simulink model "BIG_MUFF_PI_inputStage_ssc"  (R2025b)
settings: Solver=VariableStepAuto  StartTime=0  StopTime=5.1  FixedStep=1/96e3  RelTol=1e-3
libraries: fl_lib x17, ee_lib x11, nesl_utility x3
(part 2 of 2)

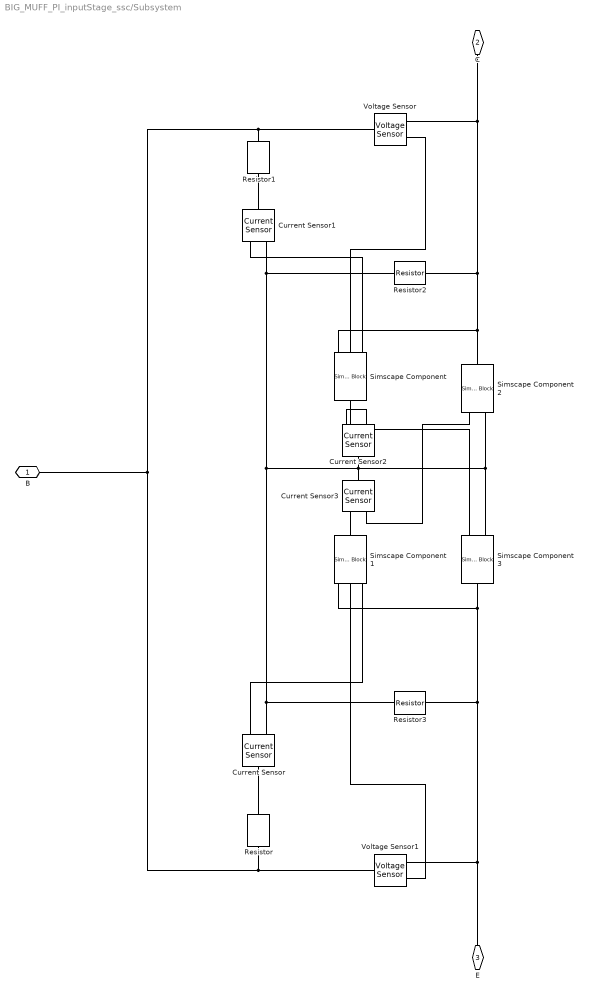
== system BIG_MUFF_PI_inputStage_ssc/Subsystem ==
  Current Sensor{,1..3} (4 alike) : fl_lib/Electrical/Electrical Sensors/Current Sensor
  Resistor : ee_lib/Passive/Resistor  R=1e-5 Ohm  enable_R_tol=0  R_tol=5  tol_distribution=1  nSigma=4  enable_operating_limits=0  operating_limit_action=2  power_rating=1 W  max_working_voltage=100 V  noise_mode=0  Tdevice=25 degC  sample_time=1e-3 s  repeatability=1  user_seed=0  auto_seed=418932850  power_derating_T1=70 degC  power_derating_T2=155 degC  operating_temperature_range_vec=[-50, 150] degC  alpha=3.93e-3 1/K  Tmeas=25 degC  thermal_mass=100 J/K  temperature_specify=off  temperature_priority=High  temperature=298.15 K  temperature_nominal_specify=off  temperature_nominal_value=1  temperature_nominal_unit=K
  Resistor1 : ee_lib/Passive/Resistor  R=1e-5 Ohm  enable_R_tol=0  R_tol=5  tol_distribution=1  nSigma=4  enable_operating_limits=0  operating_limit_action=2  power_rating=1 W  max_working_voltage=100 V  noise_mode=0  Tdevice=25 degC  sample_time=1e-3 s  repeatability=1  user_seed=0  auto_seed=1196140742  power_derating_T1=70 degC  power_derating_T2=155 degC  operating_temperature_range_vec=[-50, 150] degC  alpha=3.93e-3 1/K  Tmeas=25 degC  thermal_mass=100 J/K  temperature_specify=off  temperature_priority=High  temperature=298.15 K  temperature_nominal_specify=off  temperature_nominal_value=1  temperature_nominal_unit=K
  Resistor2 : ee_lib/Passive/Resistor  R=1e8 Ohm  enable_R_tol=0  R_tol=5  tol_distribution=1  nSigma=4  enable_operating_limits=0  operating_limit_action=2  power_rating=1 W  max_working_voltage=100 V  noise_mode=0  Tdevice=25 degC  sample_time=1e-3 s  repeatability=1  user_seed=0  auto_seed=2348838240  power_derating_T1=70 degC  power_derating_T2=155 degC  operating_temperature_range_vec=[-50, 150] degC  alpha=3.93e-3 1/K  Tmeas=25 degC  thermal_mass=100 J/K  temperature_specify=off  temperature_priority=High  temperature=298.15 K  temperature_nominal_specify=off  temperature_nominal_value=1  temperature_nominal_unit=K
  Resistor3 : ee_lib/Passive/Resistor  R=1e11 Ohm  enable_R_tol=0  R_tol=5  tol_distribution=1  nSigma=4  enable_operating_limits=0  operating_limit_action=2  power_rating=1 W  max_working_voltage=100 V  noise_mode=0  Tdevice=25 degC  sample_time=1e-3 s  repeatability=1  user_seed=0  auto_seed=4112460543  power_derating_T1=70 degC  power_derating_T2=155 degC  operating_temperature_range_vec=[-50, 150] degC  alpha=3.93e-3 1/K  Tmeas=25 degC  thermal_mass=100 J/K  temperature_specify=off  temperature_priority=High  temperature=298.15 K  temperature_nominal_specify=off  temperature_nominal_value=1  temperature_nominal_unit=K
  Simscape Component : SimscapeComponentBlock  SourceFile=bjtext_diode  ComponentPath=bjtext_diode  ComponentVariants="[\"bjtext_diode\"]"  ComponentVariantNames="[\"bjtext_diode\"]"  ClassName=bjtext_diode  SchemaVersion=1  Is=5.911e-15/0.5579 A  Rs=1e-5 V/A  eta=1  Vt=25.85e-3 V
      settings: CopyFcn=simscape.sscblock.internal.componentBlockCallback(gcbh,'COPY')  PreCopyFcn=simscape.sscblock.internal.componentBlockCallback(gcbh,'PRECOPY')  PreDeleteFcn=simscape.sscblock.internal.componentBlockCallback(gcbh,'PREDELETE')  InternalSimscapePortConfiguration="{\"Bottom\":[],\"Left\":[{\"id\":\"tail\",\"label\":\"+\",\"type\":\"foundation.electrical.electrical\"}],\"Right\":[{\"id\":\"i_in\",\"label\":\"i_in\",\"type\":\"input\"},{\"id\":\"v_in\",\"label\":\"v_in\",\"type\":\"input\"},{\"id\":\"head\",\"label\":\"-\",\"type\":\"foundation.electrical.electrical\"}],\"Top\":[]}"
      mask Type: bjtext_diode
  Simscape Component1 : SimscapeComponentBlock  SourceFile=bjtext_diode  ComponentPath=bjtext_diode  ComponentVariants="[\"bjtext_diode\"]"  ComponentVariantNames="[\"bjtext_diode\"]"  ClassName=bjtext_diode  SchemaVersion=1  Is=5.911e-15/0.9993 A  Rs=1e-5 Ohm  eta=1  Vt=25.85e-3 V
      settings: CopyFcn=simscape.sscblock.internal.componentBlockCallback(gcbh,'COPY')  PreCopyFcn=simscape.sscblock.internal.componentBlockCallback(gcbh,'PRECOPY')  PreDeleteFcn=simscape.sscblock.internal.componentBlockCallback(gcbh,'PREDELETE')  InternalSimscapePortConfiguration="{\"Bottom\":[],\"Left\":[{\"id\":\"tail\",\"label\":\"+\",\"type\":\"foundation.electrical.electrical\"}],\"Right\":[{\"id\":\"i_in\",\"label\":\"i_in\",\"type\":\"input\"},{\"id\":\"v_in\",\"label\":\"v_in\",\"type\":\"input\"},{\"id\":\"head\",\"label\":\"-\",\"type\":\"foundation.electrical.electrical\"}],\"Top\":[]}"
      mask Type: bjtext_diode
  Simscape Component2 : SimscapeComponentBlock  SourceFile=bjtext_ialpha  ComponentPath=bjtext_ialpha  ComponentVariants="[\"bjtext_ialpha\"]"  ComponentVariantNames="[\"bjtext_ialpha\"]"  ClassName=bjtext_ialpha  SchemaVersion=1  alpha=0.9993
      settings: CopyFcn=simscape.sscblock.internal.componentBlockCallback(gcbh,'COPY')  PreCopyFcn=simscape.sscblock.internal.componentBlockCallback(gcbh,'PRECOPY')  PreDeleteFcn=simscape.sscblock.internal.componentBlockCallback(gcbh,'PREDELETE')  InternalSimscapePortConfiguration="{\"Bottom\":[],\"Left\":[{\"id\":\"tail\",\"label\":\"+\",\"type\":\"foundation.electrical.electrical\"}],\"Right\":[{\"id\":\"i_in\",\"label\":\"i_in\",\"type\":\"input\"},{\"id\":\"head\",\"label\":\"-\",\"type\":\"foundation.electrical.electrical\"}],\"Top\":[]}"
      mask Type: bjtext_ialpha
  Simscape Component3 : SimscapeComponentBlock  SourceFile=bjtext_ialpha  ComponentPath=bjtext_ialpha  ComponentVariants="[\"bjtext_ialpha\"]"  ComponentVariantNames="[\"bjtext_ialpha\"]"  ClassName=bjtext_ialpha  SchemaVersion=1  alpha=0.5579
      settings: CopyFcn=simscape.sscblock.internal.componentBlockCallback(gcbh,'COPY')  PreCopyFcn=simscape.sscblock.internal.componentBlockCallback(gcbh,'PRECOPY')  PreDeleteFcn=simscape.sscblock.internal.componentBlockCallback(gcbh,'PREDELETE')  InternalSimscapePortConfiguration="{\"Bottom\":[],\"Left\":[{\"id\":\"tail\",\"label\":\"+\",\"type\":\"foundation.electrical.electrical\"}],\"Right\":[{\"id\":\"i_in\",\"label\":\"i_in\",\"type\":\"input\"},{\"id\":\"head\",\"label\":\"-\",\"type\":\"foundation.electrical.electrical\"}],\"Top\":[]}"
      mask Type: bjtext_ialpha
  Voltage Sensor : fl_lib/Electrical/Electrical Sensors/Voltage Sensor
  Voltage Sensor1 : fl_lib/Electrical/Electrical Sensors/Voltage Sensor
  B : PMIOPort  Side=Left
  C : PMIOPort  Port=2  Side=Left
  E : PMIOPort  Port=3  Side=Right
  connections:
  Voltage Sensor/RConn1 -- Simscape Component/RConn2
  Current Sensor/RConn1 -- Simscape Component1/RConn1
  Simscape Component2/LConn1 -- Resistor2/RConn1 -- Voltage Sensor/RConn2 -- C/RConn1 -- Simscape Component/RConn3
  Current Sensor3/RConn2 -- Simscape Component1/LConn1
  Current Sensor1/RConn1 -- Simscape Component/RConn1
  Resistor1/LConn1 -- Current Sensor1/LConn1
  Current Sensor2/RConn2 -- Simscape Component/LConn1
  Current Sensor/LConn1 -- Resistor/LConn1
  Voltage Sensor1/RConn1 -- Simscape Component1/RConn2
  Resistor3/RConn1 -- Simscape Component3/LConn1 -- Simscape Component1/RConn3 -- Voltage Sensor1/RConn2 -- E/RConn1
  Voltage Sensor/LConn1 -- Resistor1/RConn1 -- Resistor/RConn1 -- Voltage Sensor1/LConn1 -- B/RConn1
  Resistor2/LConn1 -- Current Sensor1/RConn2 -- Simscape Component3/RConn2 -- Simscape Component2/RConn2 -- Current Sensor3/LConn1 -- Current Sensor2/LConn1 -- Current Sensor/RConn2 -- Resistor3/LConn1
  Current Sensor2/RConn1 -- Simscape Component3/RConn1
  Current Sensor3/RConn1 -- Simscape Component2/RConn1
